simulink subsystem "Subsys_SG_Electromechanical_Part_SPS"  (R2022b)
settings: Solver=VariableStepAuto  StartTime=0.0  StopTime=10.0  RelTol=1e-3
model mask{S_n=3.2e6, f_n=50, V_n_phph=400, V_n_grid_phph=20e3, SG_Reactances=[ 3.19 0.33 0.159 1.79 0.155 0.05 ], SG_TimeConstants=[ 0.5 0.025 0.025 ], SG_StatorResistance=0.00074, SG_mech=[ 0.366 0.01 2 ], use_transformer=1, RL_Trafo_GenSide=[ 0.002 0.08 ], RL_Trafo_GridSide=[ 0.002 0.08 ], Rm_Lm=[ 500 500 ], T_s_meas=1e-4, datatype='double'}
  mask prompts: S_n "Nominal apparent power [VA]"; f_n "Nominal frequency [Hz]"; V_n_phph "Nominal SG stator voltage (rms, ph-ph) [V]"; V_n_grid_phph "Nominal grid voltage (rms, ph-ph) [V]"; SG_Reactances "Reactances [ Xd Xd' Xd'' Xq Xq'' Xl ] (pu):"; SG_TimeConstants "Time constants [ Td' Td'' Tq'' ] (s)"; SG_StatorResistance "Stator resistance (pu)"; SG_mech "Inertia, friction factor, pole pairs [ H(s) F(pu) p ]:"; use_transformer "Use transformer (0 = no, 1 = yes)"; RL_Trafo_GenSide "SG-side winding impedance [ R(pu) L(pu) ]"; RL_Trafo_GridSide "Grid-side winding impedance [ R(pu) L(pu) ]"; Rm_Lm "Magnetization resistance and inductance [ Rm(pu) Lm(pu) ]"; T_s_meas "Measurement sample time [s]"; datatype "Measurement signal data type"
undefined symbols (not defined in the file): D1, Delta
libraries: spsThreePhaseSeriesRLCLoadLib x2, spsThreePhaseVIMeasurementLib x2, spsThreePhaseBreakerLib x2, spsSynchronousMachinepuStandardLib x1, spsThreePhaseTransformerTwoWindingsLib x1
settings Model: Creator=winkens  LastModifiedBy=winkens
settings DebuggingCC: UnconnectedInputMsg=warning  UnconnectedOutputMsg=warning  UnconnectedLineMsg=warning
settings ModelReferenceCC: EnableRefExpFcnMdlSchedulingChecks=on
settings RTWCC: DLArmComputeVersion=19.05

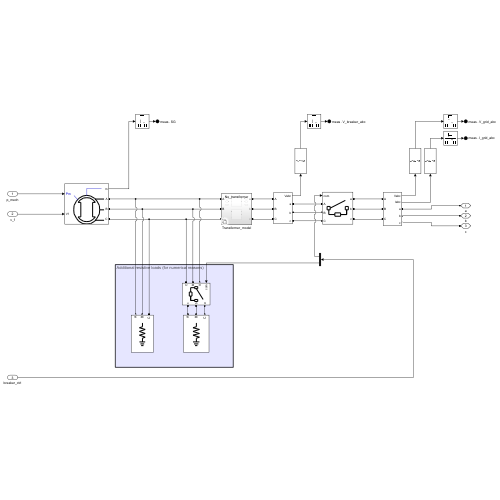
[thumbnail: Simulink's stored preview of the top-level diagram]
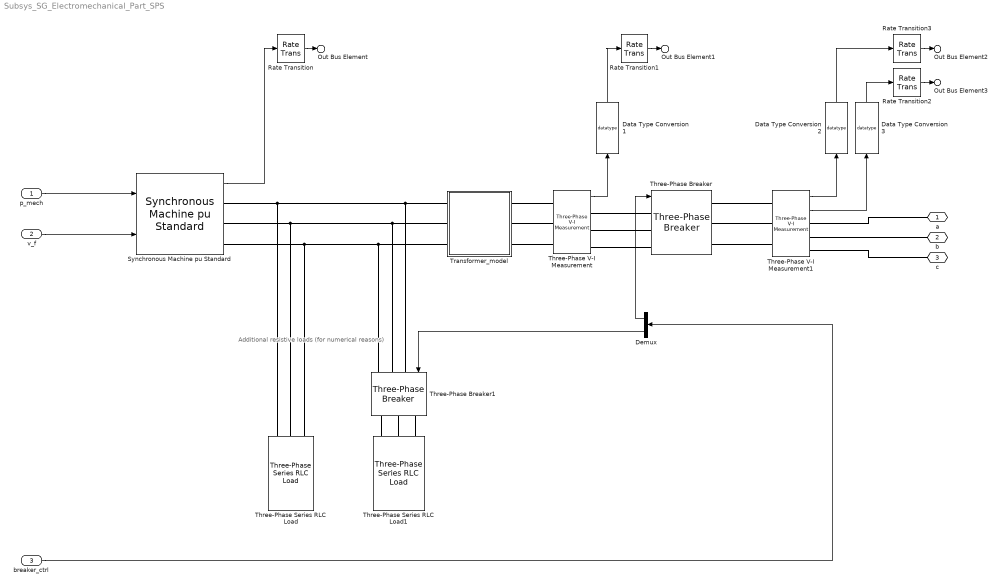
== system Subsys_SG_Electromechanical_Part_SPS ==
  note: Additional resistive loads (for numerical reasons)
  p_mech : Inport
  v_f : Inport  Port=2
  breaker_ctrl : Inport  Port=3
  Data Type Conversion1 : DataTypeConversion  OutDataTypeStr=datatype  SaturateOnIntegerOverflow=off  RndMeth=Floor
  Data Type Conversion2 : DataTypeConversion  OutDataTypeStr=datatype  SaturateOnIntegerOverflow=off  RndMeth=Floor
  Data Type Conversion3 : DataTypeConversion  OutDataTypeStr=datatype  SaturateOnIntegerOverflow=off  RndMeth=Floor
  Demux : Demux  Outputs=2
  Rate Transition{,1..3} (4 alike) : RateTransition  OutPortSampleTime=T_s_meas
  Synchronous Machine pu Standard : spsSynchronousMachinepuStandardLib/Synchronous Machine pu Standard  PresetModel=No  MechanicalLoad=Mechanical power Pm  ShowDetailedParameters=on  RotorType=Salient-pole  Units=per unit standard parameters  MeasurementBus=off  NominalParameters=[S_n V_n_phph f_n]  Reactances1=[ 1.81, 0.3, 0.23, 1.76, 0.65, 0.25, 0.15 ]  Reactances2=SG_Reactances  dAxisTimeConstants=Short-circuit  qAxisTimeConstants=Short-circuit  TimeConstants1=[2.11 0.17 0.13 1.56 0.23 0.05]  TimeConstants2=[ 8.0, 0.03, 1.0, 0.07 ]  TimeConstants3="[  4.49  0.0681  0.0513  ]"  TimeConstants4=[ 8.0, 0.03, 0.3371, 0.0295 ]  TimeConstants5=[ 1.01, 0.053, 0.1 ]  TimeConstants6=[ 1.3201, 0.023, 1.0, 0.07 ]  TimeConstants7=SG_TimeConstants  TimeConstants8=[ 1.3201, 0.0231, 0.3371, 0.0295 ]  StatorResistance=SG_StatorResistance  Mechanical=SG_mech  PolePairs=2  InitialConditions="[ 0  0  0  0  0  0  0  0  1 ]"  SetSaturation=off  Saturation=[0.6404,0.7127,0.8441,0.9214,0.9956,1.082,1.19,1.316,1.457;0.7,0.7698,0.8872,0.9466,0.9969,1.046,1.1,1.151,1.201]  LoadFlowParameters=[1,0,0,0,0]  TsPowergui=0  TsBlock=-1  IterativeModel=Trapezoidal non iterative  IterativeDiscreteModel=Trapezoidal non iterative  BusType=swing  Pref=0  Qref=0  Qmin=-inf  Qmax=inf  PLF=0  QLF=0
  Three-Phase Series RLC Load : spsThreePhaseSeriesRLCLoadLib/Three-Phase Series RLC Load  LConnTagsString=A|B|C  Configuration=Y (grounded)  NominalVoltage=V_n_phph  Vabc=[1e3 1e3 1e3]  Vabcp=[1e3 1e3 1e3]  NominalFrequency=f_n  UnbalancedPower=off  ActivePower=0.001*S_n  InductivePower=0  CapacitivePower=0  Pabc=[10e3 9e3 11e3]  QLabc=[100 90 110]  QCabc=[100 90 110]  Pabcp=[10e3 9e3 11e3]  QLabcp=[100 90 110]  QCabcp=[100 90 110]  Measurements=None  LoadType=constant Z
  Three-Phase Series RLC Load1 : spsThreePhaseSeriesRLCLoadLib/Three-Phase Series RLC Load  LConnTagsString=A|B|C  Configuration=Y (grounded)  NominalVoltage=V_n_phph  Vabc=[1e3 1e3 1e3]  Vabcp=[1e3 1e3 1e3]  NominalFrequency=f_n  UnbalancedPower=off  ActivePower=0.2*S_n  InductivePower=0  CapacitivePower=0  Pabc=[10e3 9e3 11e3]  QLabc=[100 90 110]  QCabc=[100 90 110]  Pabcp=[10e3 9e3 11e3]  QLabcp=[100 90 110]  QCabcp=[100 90 110]  Measurements=None  LoadType=constant Z
  Three-Phase V-I Measurement : spsThreePhaseVIMeasurementLib/Three-Phase V-I Measurement  VoltageMeasurement=phase-to-ground  SetLabelV=off  LabelV=Vabc  Vpu=off  VpuLL=off  CurrentMeasurement=no  SetLabelI=off  LabelI=Iabc  Ipu=off  Pbase=100e6  Vbase=500e3  OutputType=Complex  PhasorSimulation=off  PSBequivalent=0
  Three-Phase V-I Measurement1 : spsThreePhaseVIMeasurementLib/Three-Phase V-I Measurement  VoltageMeasurement=phase-to-ground  SetLabelV=off  LabelV=Vabc  Vpu=off  VpuLL=off  CurrentMeasurement=yes  SetLabelI=off  LabelI=Iabc  Ipu=off  Pbase=100e6  Vbase=500e3  OutputType=Complex  PhasorSimulation=off  PSBequivalent=0
  Three-Phase Breaker : spsThreePhaseBreakerLib/Three-Phase Breaker  InitialState=open  SwitchA=on  SwitchB=on  SwitchC=on  SwitchTimes=[]  External=on  BreakerResistance=0.01  SnubberResistance=1e6  SnubberCapacitance=inf  Measurements=None
  Three-Phase Breaker1 : spsThreePhaseBreakerLib/Three-Phase Breaker  InitialState=open  SwitchA=on  SwitchB=on  SwitchC=on  SwitchTimes=[]  External=on  BreakerResistance=0.01  SnubberResistance=1e6  SnubberCapacitance=inf  Measurements=None
  Transformer_model : Subsystem  Variant=on  VariantControl=Choice
  a : PMIOPort  Side=Right
  b : PMIOPort  Port=2  Side=Right
  c : PMIOPort  Port=3  Side=Right
  Out Bus Element : Outport  PortName=meas  Element=SG
  Out Bus Element1 : Outport  PortName=meas  Element=V_breaker_abc
  Out Bus Element2 : Outport  PortName=meas  Element=V_grid_abc
  Out Bus Element3 : Outport  PortName=meas  Element=I_grid_abc
  wires:
  Three-Phase V-I Measurement/1 -> Data Type Conversion1/1
  p_mech/1 -> Synchronous Machine pu Standard/1
  Three-Phase V-I Measurement1/2 -> Data Type Conversion3/1
  breaker_ctrl/1 -> Demux/1
  Demux/1 -> Three-Phase Breaker/1
  Demux/2 -> Three-Phase Breaker1/1
  v_f/1 -> Synchronous Machine pu Standard/2
  Three-Phase V-I Measurement1/1 -> Data Type Conversion2/1
  Rate Transition/1 -> Out Bus Element/1
  Rate Transition1/1 -> Out Bus Element1/1
  Rate Transition2/1 -> Out Bus Element3/1
  Rate Transition3/1 -> Out Bus Element2/1
  Synchronous Machine pu Standard/1 -> Rate Transition/1
  Data Type Conversion1/1 -> Rate Transition1/1
  Data Type Conversion2/1 -> Rate Transition3/1
  Data Type Conversion3/1 -> Rate Transition2/1
  connections:
  Three-Phase Breaker1/LConn3 -- Synchronous Machine pu Standard/RConn3 -- Three-Phase Series RLC Load/LConn3 -- Transformer_model/LConn3
  Three-Phase Breaker1/LConn2 -- Synchronous Machine pu Standard/RConn2 -- Three-Phase Series RLC Load/LConn2 -- Transformer_model/LConn2
  Three-Phase Breaker1/LConn1 -- Synchronous Machine pu Standard/RConn1 -- Three-Phase Series RLC Load/LConn1 -- Transformer_model/LConn1
  Three-Phase V-I Measurement/RConn3 -- Three-Phase Breaker/LConn3
  Three-Phase Series RLC Load1/LConn1 -- Three-Phase Breaker1/RConn3
  Three-Phase Series RLC Load1/LConn3 -- Three-Phase Breaker1/RConn1
  Three-Phase V-I Measurement/RConn1 -- Three-Phase Breaker/LConn1
  Three-Phase V-I Measurement1/RConn2 -- b/RConn1
  Three-Phase Series RLC Load1/LConn2 -- Three-Phase Breaker1/RConn2
  Three-Phase Breaker/RConn1 -- Three-Phase V-I Measurement1/LConn1
  Three-Phase Breaker/RConn2 -- Three-Phase V-I Measurement1/LConn2
  Three-Phase V-I Measurement/RConn2 -- Three-Phase Breaker/LConn2
  Three-Phase Breaker/RConn3 -- Three-Phase V-I Measurement1/LConn3
  Three-Phase V-I Measurement1/RConn1 -- a/RConn1
  Three-Phase V-I Measurement1/RConn3 -- c/RConn1
  Transformer_model/RConn1 -- Three-Phase V-I Measurement/LConn1
  Transformer_model/RConn2 -- Three-Phase V-I Measurement/LConn2
  Transformer_model/RConn3 -- Three-Phase V-I Measurement/LConn3

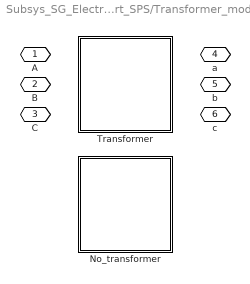
== system Subsys_SG_Electromechanical_Part_SPS/Transformer_model ==
  No_transformer : Subsystem  VariantControl=use_transformer == 0
  Transformer : Subsystem  VariantControl=(default)
  A : PMIOPort  Side=Left
  B : PMIOPort  Port=2  Side=Left
  C : PMIOPort  Port=3  Side=Left
  a : PMIOPort  Port=4  Side=Right
  b : PMIOPort  Port=5  Side=Right
  c : PMIOPort  Port=6  Side=Right

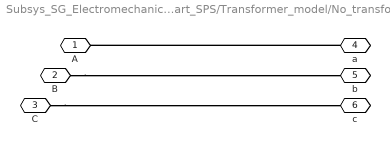
== system Subsys_SG_Electromechanical_Part_SPS/Transformer_model/No_transformer ==
  A : PMIOPort  Side=Left
  B : PMIOPort  Port=2  Side=Left
  C : PMIOPort  Port=3  Side=Left
  a : PMIOPort  Port=4  Side=Right
  b : PMIOPort  Port=5  Side=Right
  c : PMIOPort  Port=6  Side=Right
  connections:
  B/RConn1 -- b/RConn1
  C/RConn1 -- c/RConn1
  a/RConn1 -- A/RConn1

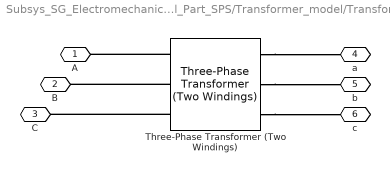
== system Subsys_SG_Electromechanical_Part_SPS/Transformer_model/Transformer ==
  Three-Phase Transformer (Two Windings) : spsThreePhaseTransformerTwoWindingsLib/Three-Phase Transformer (Two Windings)  Winding1Connection=Delta (D1)  Winding2Connection=Delta (D1)  CoreType=Three-limb core (core-type)  SetSaturation=off  Hysteresis=off  DataFile='hysteresis'  SetInitialFlux=off  Measurements=None  UNITS=pu  NominalPower=[ S_n , f_n ]  Winding1=[ V_n_phph , RL_Trafo_GenSide(1) , RL_Trafo_GenSide(2) ]  Winding2=[ V_n_grid_phph , RL_Trafo_GridSide(1) , RL_Trafo_GridSide(2) ]  Rm=Rm_Lm(1)  Lm=Rm_Lm(2)  L0=0.5  Saturation=[ 0,0 ; 0.0024,1.2 ; 1.0,1.52 ]  InitialFluxes=[ 0.8 , -0.8 , 0.7 ]  BreakLoop=off  DiscreteSolver=Trapezoidal iterative  DataType=off  TransfoNumber=1
  A : PMIOPort  Side=Left
  B : PMIOPort  Port=2  Side=Left
  C : PMIOPort  Port=3  Side=Left
  a : PMIOPort  Port=4  Side=Right
  b : PMIOPort  Port=5  Side=Right
  c : PMIOPort  Port=6  Side=Right
  connections:
  Three-Phase Transformer (Two Windings)/RConn2 -- b/RConn1
  Three-Phase Transformer (Two Windings)/RConn3 -- c/RConn1
  Three-Phase Transformer (Two Windings)/LConn1 -- A/RConn1
  Three-Phase Transformer (Two Windings)/RConn1 -- a/RConn1
  Three-Phase Transformer (Two Windings)/LConn2 -- B/RConn1
  Three-Phase Transformer (Two Windings)/LConn3 -- C/RConn1
